simulink model "plant"  (R2025a)
settings: Solver=FixedStepAuto  StartTime=0.0  StopTime=10.0  FixedStep=0.005  MaxStep=0.2  RelTol=1e-3
InitFcn:
  | script
model workspace (MATLAB code in the model file):
  | script
values from neighbouring files (symbols this model uses):
  A = [0, 1, 0, 0 ... (first row only)    [control_synthesis.m]
  A_obs = [0, 1, 0 ... (first row only)    [control_synthesis.m]
  B = [0; N \ B_b]    [control_synthesis.m]
  B_obs = [-d_i, 0 ... (first row only)    [control_synthesis.m]
  C_obs = [1 / rho, 0, -1]    [control_synthesis.m]
  d_i = 0.180    (= 0.18)    [control_synthesis.m]
  g = 9.81    [control_synthesis.m]
  L_obs = place(A_obs', C_obs', observer_poles)'    [control_synthesis.m]
undefined symbols (not defined in the file or in its folder): K
settings Model: Creator=elyes  LastModifiedBy=elyes

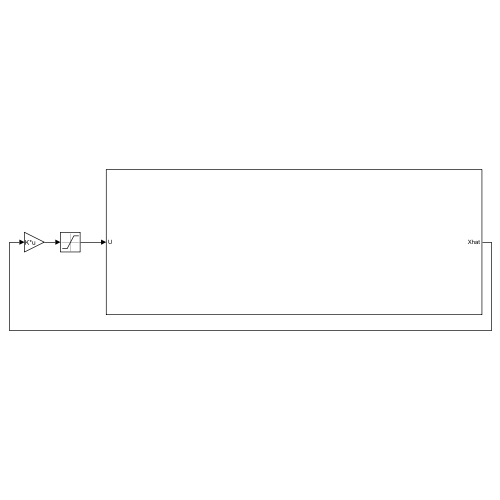
[thumbnail: Simulink's stored preview of the top-level diagram]
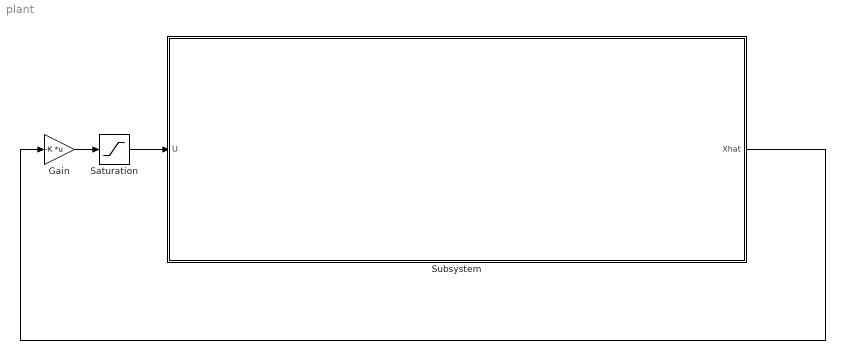
== system plant ==
  Gain : Gain  Gain=-K  Multiplication=Matrix(K*u)
  Saturation : Saturate  UpperLimit=24  LowerLimit=-24
  Subsystem : Subsystem
  wires:
  Gain/1 -> Saturation/1
  Subsystem/1(Xhat) -> Gain/1
  Saturation/1 -> Subsystem/1(U)

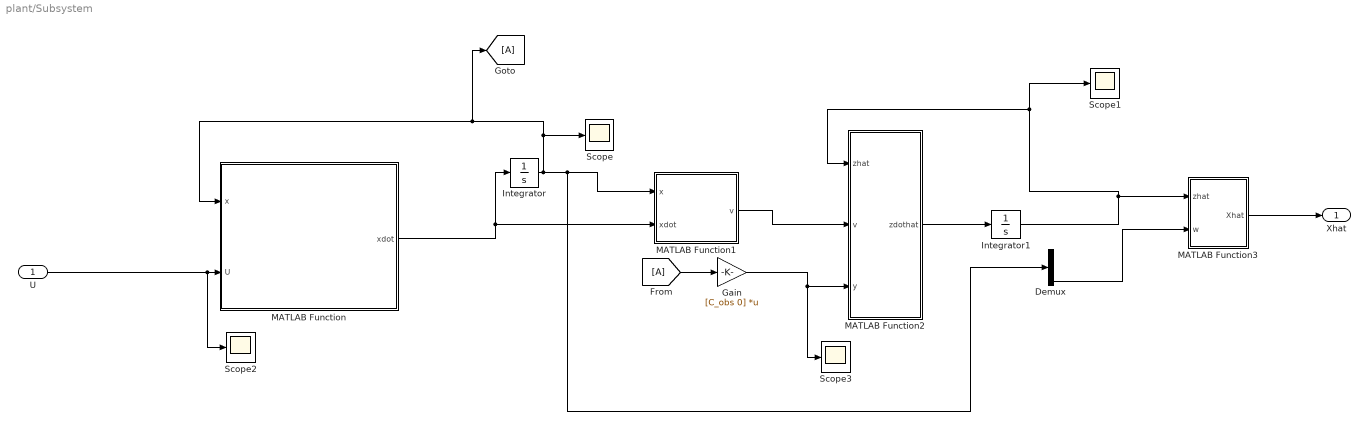
== system plant/Subsystem ==
  U : Inport
  Demux : Demux
  From : From
  Gain : Gain  Gain=[C_obs 0]  Multiplication=Matrix(K*u)
  Goto : Goto
  Integrator : Integrator  InitialCondition=[0.;0;0.01;0]
  Integrator1 : Integrator  InitialCondition=[0;0;0.01]
  MATLAB Function : MATLAB Function  TreatAsAtomicUnit=on
  MATLAB Function1 : MATLAB Function  TreatAsAtomicUnit=on
  MATLAB Function2 : MATLAB Function  TreatAsAtomicUnit=on
  MATLAB Function3 : MATLAB Function  TreatAsAtomicUnit=on
  Scope{,1..3} (4 alike) : Scope
      Scope settings: ActiveDisplayYMinimum=-0.065269848792287047  ActiveDisplayYMaximum=0.037664979200419287
      Scope1 settings: ActiveDisplayYMinimum=-0.0048119329111651985  ActiveDisplayYMaximum=0.020095178402998067
      Scope2 settings: ActiveDisplayYMinimum=-0.10658523239451223  ActiveDisplayYMaximum=0.63890817294236446  DataLoggingVariableName=ScopeData2
      Scope3 settings: ActiveDisplayYMinimum=-85649.90794832223  ActiveDisplayYMaximum=9567.7774411568134  DataLoggingVariableName=ScopeData3
  Xhat : Outport  PortDimensions=4
  wires:
  MATLAB Function1/1(v) -> MATLAB Function2/2(v)
  Integrator1/1 -> Scope1/1, MATLAB Function2/1(zhat), MATLAB Function3/1(zhat)
  MATLAB Function2/1(zdothat) -> Integrator1/1
  MATLAB Function/1(xdot) -> Integrator/1, MATLAB Function1/2(xdot)
  U/1 -> Scope2/1, MATLAB Function/2(U)
  Gain/1 -> Scope3/1, MATLAB Function2/3(y)
  From/1 -> Gain/1
  Demux/4 -> MATLAB Function3/2(w)
  Integrator/1 -> Goto/1, MATLAB Function/1(x), Scope/1, Demux/1, MATLAB Function1/1(x)
  MATLAB Function3/1(Xhat) -> Xhat/1

== matlab function plant/Subsystem/MATLAB Function1 ==
  data: x input; v output; xdot input; d_i parameter; g parameter
function v = fcn(x,xdot,d_i, g)

v = zeros(2,1);
v(1) = x(4);
v(2) = xdot(2)+d_i*xdot(4)-g*x(3);

== matlab function plant/Subsystem/MATLAB Function ==
  data: x input; xdot output; U input; A parameter; B parameter
function xdot= fcn(x,U,A,B)

xdot = A*x + B*U;

== matlab function plant/Subsystem/MATLAB Function2 ==
  data: zhat input; v input; y input; zdothat output; A_obs parameter; B_obs parameter; C_obs parameter; L_obs parameter
function zdothat = fcn(zhat,v,y,A_obs, B_obs, C_obs, L_obs)

zdothat = A_obs*zhat + B_obs*v + L_obs*(y-C_obs*zhat);

== matlab function plant/Subsystem/MATLAB Function3 ==
  data: zhat input; Xhat output; w input; d_i parameter
function Xhat = fcn(zhat,w, d_i)

Xhat = zeros(4,1);
Xhat(1) = zhat(1);
Xhat(2) = zhat(2) - d_i * w;
Xhat(3) = zhat(3);
Xhat(4) = w;
